simulink model "system_ident_model"  (R2025b)
settings: Solver=FixedStepAuto  StartTime=0.0  StopTime=t_f  FixedStep=t_s  RelTol=1e-3
values from neighbouring files (symbols this model uses):
  denom = [I*L I*R (L*c + k_f*k_e*r^2)  R*c]    [system_init.m]
  k_enc = 4096 / (2 * pi)    (= 651.898646904)    [system_init.m]
  nom = r*k_f    (= 0.73794)    [system_init.m]
  r_2 = r    (= 0.1004)    [system_init.m]
  t_fs = t_f/N_p    (= 20)    [system_init.m]
  t_s = 0.0005    [system_init.m]
  V_max = 60    [system_init.m]
  w_0 = 1e-3    (= 0.001)    [system_init.m]
  w_f = 1e3    (= 1000)    [system_init.m]
settings Model: Creator=KnaZ  LastModifiedBy=KnaZ

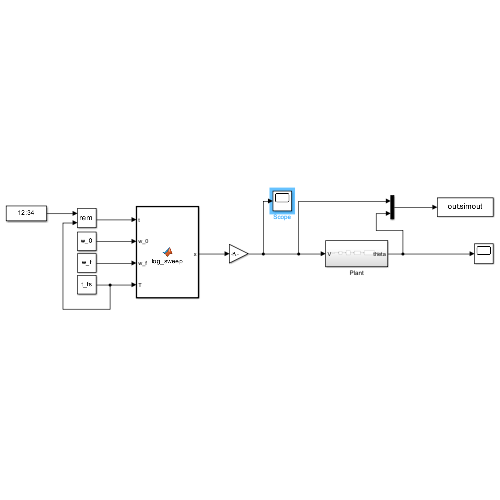
[thumbnail: Simulink's stored preview of the top-level diagram]
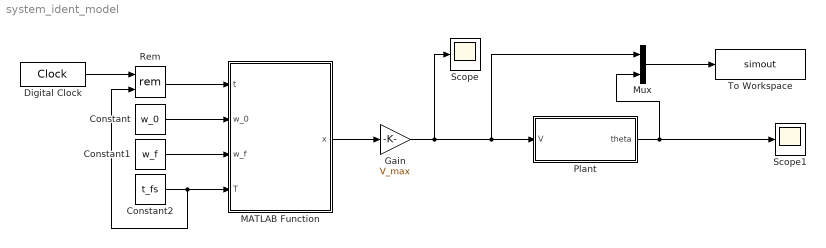
== system system_ident_model ==
  Constant : Constant  Value=w_0
  Constant1 : Constant  Value=w_f
  Constant2 : Constant  Value=t_fs
  Digital Clock : DigitalClock  SampleTime=t_s
  Gain : Gain  Gain=V_max
  MATLAB Function : MATLAB Function  TreatAsAtomicUnit=on
  Mux : Mux  Inputs=2
  Plant : Subsystem
  Rem : Math  Operator=rem
  Scope : Scope
      settings: ActiveDisplayYMinimum=-107.21345914105555  ActiveDisplayYMaximum=114.13135318705358
  Scope1 : Scope
      settings: ActiveDisplayYMinimum=-0.015566392602506774  ActiveDisplayYMaximum=0.015691872379484502
  To Workspace : ToWorkspace  VariableName=simout  SaveFormat=Structure With Time  SampleTime=-1
  wires:
  Constant/1 -> MATLAB Function/2(w_0)
  Constant1/1 -> MATLAB Function/3(w_f)
  Constant2/1 -> Rem/2, MATLAB Function/4(T)
  Mux/1 -> To Workspace/1
  MATLAB Function/1(x) -> Gain/1
  Gain/1 -> Scope/1, Plant/1(V), Mux/1
  Rem/1 -> MATLAB Function/1(t)
  Digital Clock/1 -> Rem/1
  Plant/1(theta) -> Scope1/1, Mux/2

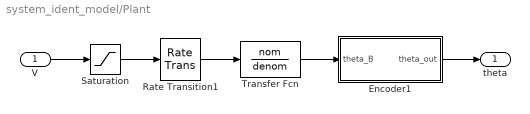
== system system_ident_model/Plant ==
  V : Inport
  Encoder1 : Subsystem
  Rate Transition1 : RateTransition  OutPortSampleTime=0
  Saturation : Saturate  UpperLimit=V_max  LowerLimit=-V_max
  Transfer Fcn : TransferFcn  Numerator=nom  Denominator=denom
  theta : Outport
  wires:
  Transfer Fcn/1 -> Encoder1/1(theta_B)
  Rate Transition1/1 -> Transfer Fcn/1
  Saturation/1 -> Rate Transition1/1
  V/1 -> Saturation/1
  Encoder1/1(theta_out) -> theta/1

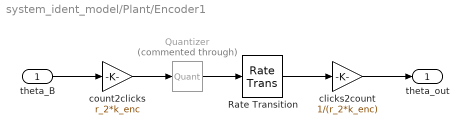
== system system_ident_model/Plant/Encoder1 ==
  theta_B : Inport
  Quantizer : Quantizer  Commented=through  QuantizationInterval=1
  Rate Transition : RateTransition  OutPortSampleTime=t_s
  clicks2count : Gain  Gain=1/(r_2*k_enc)
  count2clicks : Gain  Gain=r_2*k_enc
  theta_out : Outport
  wires:
  theta_B/1 -> count2clicks/1
  Rate Transition/1 -> clicks2count/1
  clicks2count/1 -> theta_out/1
  count2clicks/1 -> Quantizer/1
  Quantizer/1 -> Rate Transition/1

== matlab function system_ident_model/MATLAB Function ==
  data: t input; x output; w_0 input; w_f input; T input
function x = log_sweep(t, w_0, w_f, T)
    K = w_0 * T / log(w_f / w_0);
    L = T / log(w_f / w_0);

    x = sin(K .* (exp(t ./ L) - 1));
end
